simulink model "SoftGripperPick"  (R2026b)
settings: Solver=daessc  StopTime=16  RelTol=1e-4
undefined symbols (not defined in the file): magnitude, P, X, Y, Z
libraries: sm_lib x123, nesl_utility x40, fl_lib x4
(part 1 of 3)
settings Model: Creator=amavromm  LastModifiedBy=amavromm
settings SolverCC: ZeroCrossControl=DisableAll
settings SimscapeCC: SimscapeNominalValues="[{\"value\":\"1\",\"unit\":\"A\"},{\"value\":\"1\",\"unit\":\"bar\"},{\"value\":\"1\",\"unit\":\"cm^2\"},{\"value\":\"1\",\"unit\":\"cm^3/s\"},{\"value\":\"1\",\"unit\":\"kJ/kg\"},{\"value\":\"1\",\"unit\":\"kW\"},{\"value\":\"1\",\"unit\":\"l\"},{\"value\":\"1\",\"unit\":\"N\"},{\"value\":\"1\",\"unit\":\"N*m\"},{\"value\":\"1\",\"unit\":\"V\"},{\"value\":\"0.001\",\"unit\":\"Wb\"}]"  SimscapeUseEnergyAccounting=off

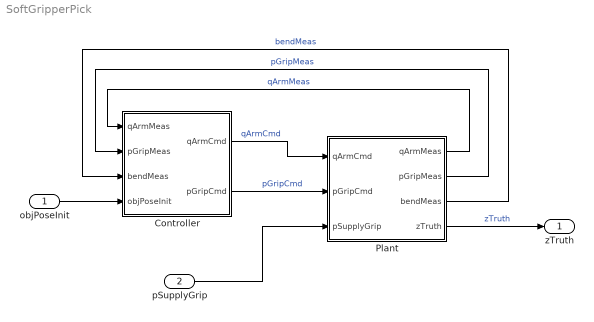
== system SoftGripperPick ==
  objPoseInit : Inport  PortDimensions=6
  pSupplyGrip : Inport  Port=2  PortDimensions=1
  Controller : Subsystem
  Plant : Subsystem
  zTruth : Outport
  wires:
  Plant/4(zTruth) -> zTruth/1  "zTruth"
  objPoseInit/1 -> Controller/4(objPoseInit)
  Plant/3(bendMeas) -> Controller/3(bendMeas)  "bendMeas"
  Plant/2(pGripMeas) -> Controller/2(pGripMeas)  "pGripMeas"
  Plant/1(qArmMeas) -> Controller/1(qArmMeas)  "qArmMeas"
  pSupplyGrip/1 -> Plant/3(pSupplyGrip)
  Controller/2(pGripCmd) -> Plant/2(pGripCmd)  "pGripCmd"
  Controller/1(qArmCmd) -> Plant/1(qArmCmd)  "qArmCmd"

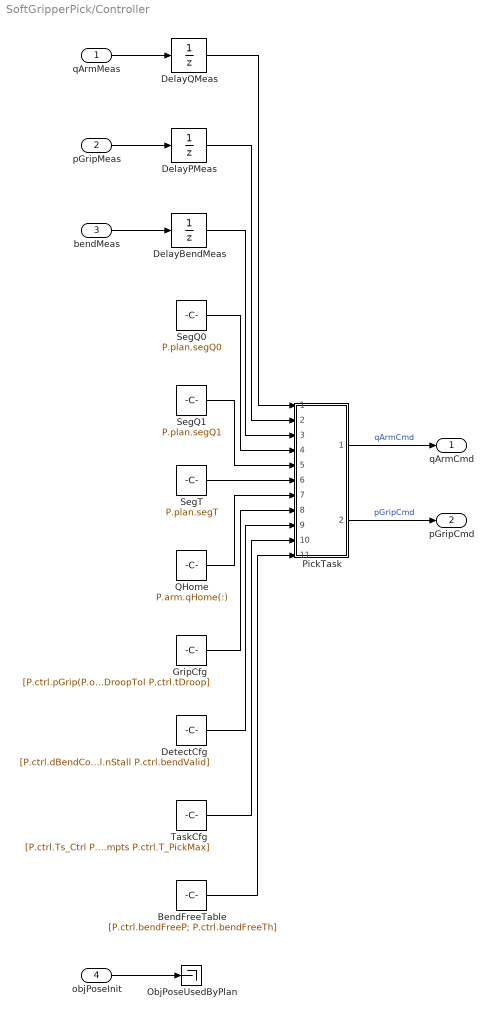
== system SoftGripperPick/Controller ==
  qArmMeas : Inport
  pGripMeas : Inport  Port=2
  bendMeas : Inport  Port=3
  objPoseInit : Inport  Port=4
  BendFreeTable : Constant  Value=[P.ctrl.bendFreeP; P.ctrl.bendFreeTh]
  DelayBendMeas : UnitDelay  InitialCondition=zeros(4,1)  SampleTime=P.ctrl.Ts_Ctrl
  DelayPMeas : UnitDelay  SampleTime=P.ctrl.Ts_Ctrl
  DelayQMeas : UnitDelay  InitialCondition=P.arm.qHome(:)  SampleTime=P.ctrl.Ts_Ctrl
  DetectCfg : Constant  Value=[P.ctrl.dBendContact P.ctrl.stallRate P.ctrl.nStall P.ctrl.bendValid]
  GripCfg : Constant  Value=[P.ctrl.pGrip(P.objId) P.ctrl.sens.pAcc P.ctrl.tCloseRamp P.ctrl.tCloseMax P.ctrl.tVent P.ctrl.pDroopTol P.ctrl.tDroop]
  ObjPoseUsedByPlan : Terminator
  PickTask : Stateflow chart  TreatAsAtomicUnit=on
  QHome : Constant  Value=P.arm.qHome(:)
  SegQ0 : Constant  Value=P.plan.segQ0
  SegQ1 : Constant  Value=P.plan.segQ1
  SegT : Constant  Value=P.plan.segT
  TaskCfg : Constant  Value=[P.ctrl.Ts_Ctrl P.ctrl.tSettle P.ctrl.qTol P.ctrl.N_Attempts P.ctrl.T_PickMax]
  qArmCmd : Outport
  pGripCmd : Outport  Port=2
  wires:
  DelayBendMeas/1 -> PickTask/3(bend)
  DelayPMeas/1 -> PickTask/2(pMeas)
  DelayQMeas/1 -> PickTask/1(qMeas)
  objPoseInit/1 -> ObjPoseUsedByPlan/1
  qArmMeas/1 -> DelayQMeas/1
  pGripMeas/1 -> DelayPMeas/1
  bendMeas/1 -> DelayBendMeas/1
  SegQ0/1 -> PickTask/4(segQ0)
  SegQ1/1 -> PickTask/5(segQ1)
  SegT/1 -> PickTask/6(segT)
  QHome/1 -> PickTask/7(qHome)
  GripCfg/1 -> PickTask/8(gripCfg)
  DetectCfg/1 -> PickTask/9(detCfg)
  TaskCfg/1 -> PickTask/10(taskCfg)
  BendFreeTable/1 -> PickTask/11(bendTab)
  PickTask/1(qCmd) -> qArmCmd/1  "qArmCmd"
  PickTask/2(pCmd) -> pGripCmd/1  "pGripCmd"

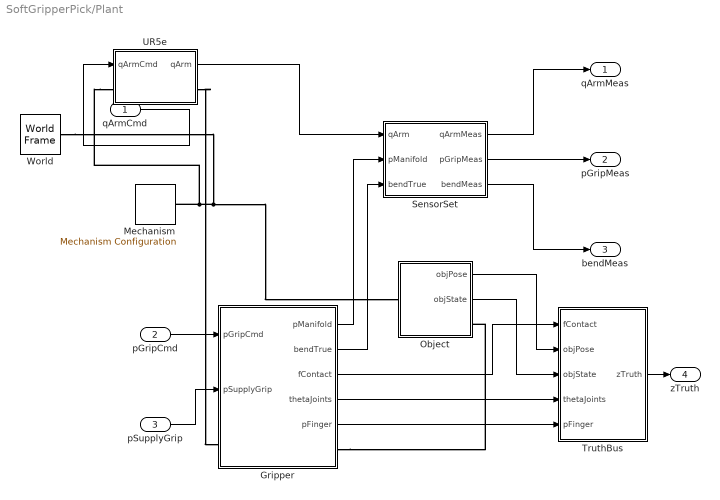
== system SoftGripperPick/Plant ==
  qArmCmd : Inport
  pGripCmd : Inport  Port=2
  pSupplyGrip : Inport  Port=3
  Gripper : Subsystem
  Mechanism : sm_lib/Utilities/Mechanism Configuration  UniformGravity=Constant  GravityVector=[0 0 -9.80665]  GravityVectorUnits=m/s^2  LinearizationDelta=0.001  JointModeTransitionNonlinearIterations=2
  Object : Subsystem
  SensorSet : Subsystem
  TruthBus : Subsystem
  UR5e : Subsystem
  World : sm_lib/Frames and Transforms/World Frame
  qArmMeas : Outport
  pGripMeas : Outport  Port=2
  bendMeas : Outport  Port=3
  zTruth : Outport  Port=4
  wires:
  Gripper/5(pFinger) -> TruthBus/5(pFinger)
  Gripper/4(thetaJoints) -> TruthBus/4(thetaJoints)
  Gripper/3(fContact) -> TruthBus/1(fContact)
  Gripper/2(bendTrue) -> SensorSet/3(bendTrue)
  Gripper/1(pManifold) -> SensorSet/2(pManifold)
  UR5e/1(qArm) -> SensorSet/1(qArm)
  pSupplyGrip/1 -> Gripper/2(pSupplyGrip)
  pGripCmd/1 -> Gripper/1(pGripCmd)
  qArmCmd/1 -> UR5e/1(qArmCmd)
  SensorSet/1(qArmMeas) -> qArmMeas/1
  SensorSet/2(pGripMeas) -> pGripMeas/1
  SensorSet/3(bendMeas) -> bendMeas/1
  Object/1(objPose) -> TruthBus/2(objPose)
  Object/2(objState) -> TruthBus/3(objState)
  TruthBus/1(zTruth) -> zTruth/1
  connections:
  UR5e/LConn1 -- World/RConn1 -- Object/LConn1 -- Mechanism/RConn1
  Gripper/RConn1 -- Object/RConn1
  UR5e/RConn1 -- Gripper/LConn1

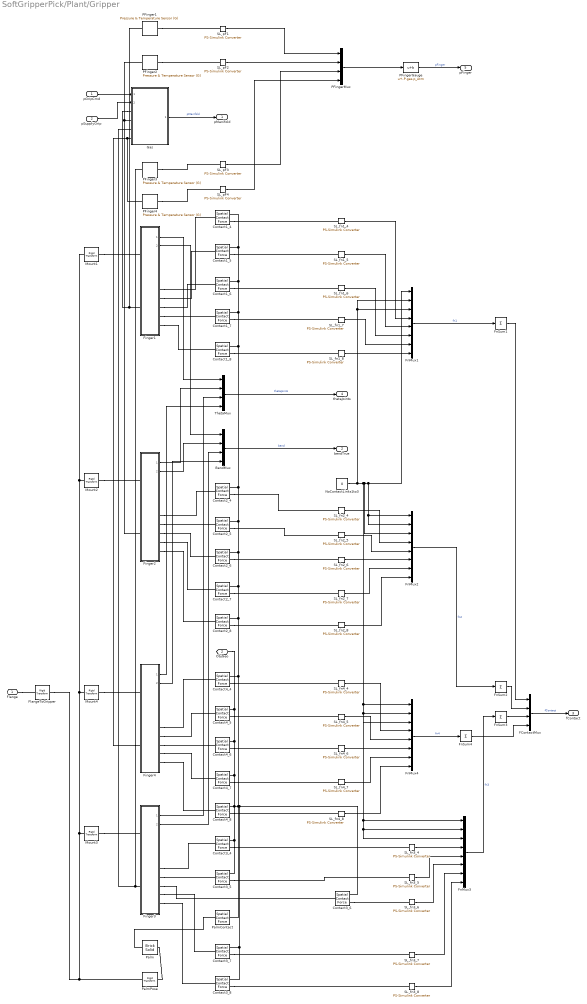
== system SoftGripperPick/Plant/Gripper ==
  pGripCmd : Inport
  pSupplyGrip : Inport  Port=2
  BendMux : Mux
  Contact1_{4..8} (5 alike) : sm_lib/Forces and Torques/Spatial Contact Force  SenseSeparationDistance=off  NormalForceType=SmoothSpringDamper  NormalStiffness=P.obj.k_Contact  NormalStiffnessUnits=N/m  NormalDamping=P.obj.c_Contact  NormalDampingUnits=N/(m/s)  NormalTransitionRegionWidth=P.bench.wContact  NormalTransitionRegionWidthUnits=m  FrictionType=SmoothStickSlip  CoefficientOfStaticFriction=P.obj.mu_s  CoefficientOfDynamicFriction=P.obj.mu_d  FrictionalCriticalVelocity=P.bench.vCrit  FrictionalCriticalVelocityUnits=m/s  SenseContactSignal=off  SensePenetrationDepth=off  SenseNormalVelocity=off  SenseTangentialVelocity=off  SensingForceTorqueDirection=BaseOnFollower  SensingForceTorqueResolutionFrame=ContactFrame  SenseNormalForce=off  SenseNormalForceMagnitude=on  SenseNormalTorque=off  SenseFrictionalForce=off  SenseFrictionalForceMagnitude=off  SenseFrictionalTorque=off  SenseTotalForce=off  SenseTotalTorque=off  SenseContactBaseRotation=off  SenseContactBaseTranslation=off  SenseContactFollowerRotation=off  SenseContactFollowerTranslation=off  ZeroCrossDetectContactStartAndEnd=off
  Contact2_{4..8} (5 alike) : sm_lib/Forces and Torques/Spatial Contact Force  SenseSeparationDistance=off  NormalForceType=SmoothSpringDamper  NormalStiffness=P.obj.k_Contact  NormalStiffnessUnits=N/m  NormalDamping=P.obj.c_Contact  NormalDampingUnits=N/(m/s)  NormalTransitionRegionWidth=P.bench.wContact  NormalTransitionRegionWidthUnits=m  FrictionType=SmoothStickSlip  CoefficientOfStaticFriction=P.obj.mu_s  CoefficientOfDynamicFriction=P.obj.mu_d  FrictionalCriticalVelocity=P.bench.vCrit  FrictionalCriticalVelocityUnits=m/s  SenseContactSignal=off  SensePenetrationDepth=off  SenseNormalVelocity=off  SenseTangentialVelocity=off  SensingForceTorqueDirection=BaseOnFollower  SensingForceTorqueResolutionFrame=ContactFrame  SenseNormalForce=off  SenseNormalForceMagnitude=on  SenseNormalTorque=off  SenseFrictionalForce=off  SenseFrictionalForceMagnitude=off  SenseFrictionalTorque=off  SenseTotalForce=off  SenseTotalTorque=off  SenseContactBaseRotation=off  SenseContactBaseTranslation=off  SenseContactFollowerRotation=off  SenseContactFollowerTranslation=off  ZeroCrossDetectContactStartAndEnd=off
  Contact3_{4..8} (5 alike) : sm_lib/Forces and Torques/Spatial Contact Force  SenseSeparationDistance=off  NormalForceType=SmoothSpringDamper  NormalStiffness=P.obj.k_Contact  NormalStiffnessUnits=N/m  NormalDamping=P.obj.c_Contact  NormalDampingUnits=N/(m/s)  NormalTransitionRegionWidth=P.bench.wContact  NormalTransitionRegionWidthUnits=m  FrictionType=SmoothStickSlip  CoefficientOfStaticFriction=P.obj.mu_s  CoefficientOfDynamicFriction=P.obj.mu_d  FrictionalCriticalVelocity=P.bench.vCrit  FrictionalCriticalVelocityUnits=m/s  SenseContactSignal=off  SensePenetrationDepth=off  SenseNormalVelocity=off  SenseTangentialVelocity=off  SensingForceTorqueDirection=BaseOnFollower  SensingForceTorqueResolutionFrame=ContactFrame  SenseNormalForce=off  SenseNormalForceMagnitude=on  SenseNormalTorque=off  SenseFrictionalForce=off  SenseFrictionalForceMagnitude=off  SenseFrictionalTorque=off  SenseTotalForce=off  SenseTotalTorque=off  SenseContactBaseRotation=off  SenseContactBaseTranslation=off  SenseContactFollowerRotation=off  SenseContactFollowerTranslation=off  ZeroCrossDetectContactStartAndEnd=off
  Contact4_{4..8} (5 alike) : sm_lib/Forces and Torques/Spatial Contact Force  SenseSeparationDistance=off  NormalForceType=SmoothSpringDamper  NormalStiffness=P.obj.k_Contact  NormalStiffnessUnits=N/m  NormalDamping=P.obj.c_Contact  NormalDampingUnits=N/(m/s)  NormalTransitionRegionWidth=P.bench.wContact  NormalTransitionRegionWidthUnits=m  FrictionType=SmoothStickSlip  CoefficientOfStaticFriction=P.obj.mu_s  CoefficientOfDynamicFriction=P.obj.mu_d  FrictionalCriticalVelocity=P.bench.vCrit  FrictionalCriticalVelocityUnits=m/s  SenseContactSignal=off  SensePenetrationDepth=off  SenseNormalVelocity=off  SenseTangentialVelocity=off  SensingForceTorqueDirection=BaseOnFollower  SensingForceTorqueResolutionFrame=ContactFrame  SenseNormalForce=off  SenseNormalForceMagnitude=on  SenseNormalTorque=off  SenseFrictionalForce=off  SenseFrictionalForceMagnitude=off  SenseFrictionalTorque=off  SenseTotalForce=off  SenseTotalTorque=off  SenseContactBaseRotation=off  SenseContactBaseTranslation=off  SenseContactFollowerRotation=off  SenseContactFollowerTranslation=off  ZeroCrossDetectContactStartAndEnd=off
  FContactMux : Mux
  Finger{1..4} (4 alike) : Subsystem  ReferencedSubsystem=SoftFinger
  FlangeToGripper : sm_lib/Frames and Transforms/Rigid Transform  RotationMethod=StandardAxis  FollAlignAxisA=+X  BaseAlignAxisA=+Y  FollAlignAxisB=+Y  BaseAlignAxisB=+Z  RotationStandardAxis=+X  RotationAngle=180  RotationAngleUnits=deg  RotationArbitraryAxis=[0 0 1]  RotationSequenceAxes=FollowerAxes  RotationSequence=XYX  RotationSequenceAngles=[0 0 0]  RotationSequenceAnglesUnits=deg  RotationMatrix=[1 0 0;0 1 0;0 0 1]  Quaternion=[1 0 0 0]  TranslationMethod=None  TranslationCartesianOffset=[0 0 0]  TranslationCartesianOffsetUnits=m  TranslationStandardAxis=+Z  TranslationStandardOffset=0  TranslationStandardOffsetUnits=m  TranslationROffset=0  TranslationROffsetUnits=m  TranslationThetaOffset=0  TranslationThetaOffsetUnits=deg  TranslationZOffset=0  TranslationZOffsetUnits=m
  FnMux{1..4} (4 alike) : Mux  Inputs=8
  FnSum{1..4} (4 alike) : Sum  Inputs=+
  Gas : Subsystem  ReferencedSubsystem=GripperGas
  Mount1 : sm_lib/Frames and Transforms/Rigid Transform  RotationMethod=RotationMatrix  FollAlignAxisA=+X  BaseAlignAxisA=+Y  FollAlignAxisB=+Y  BaseAlignAxisB=+Z  RotationStandardAxis=+Z  RotationAngle=0  RotationAngleUnits=deg  RotationArbitraryAxis=[0 0 1]  RotationSequenceAxes=FollowerAxes  RotationSequence=XYX  RotationSequenceAngles=[0 0 0]  RotationSequenceAnglesUnits=deg  RotationMatrix=P.bench.mountR(:,:,1)  Quaternion=[1 0 0 0]  TranslationMethod=Cartesian  TranslationCartesianOffset=P.bench.mountT(1,:)  TranslationCartesianOffsetUnits=m  TranslationStandardAxis=+Z  TranslationStandardOffset=0  TranslationStandardOffsetUnits=m  TranslationROffset=0  TranslationROffsetUnits=m  TranslationThetaOffset=0  TranslationThetaOffsetUnits=deg  TranslationZOffset=0  TranslationZOffsetUnits=m
  Mount2 : sm_lib/Frames and Transforms/Rigid Transform  RotationMethod=RotationMatrix  FollAlignAxisA=+X  BaseAlignAxisA=+Y  FollAlignAxisB=+Y  BaseAlignAxisB=+Z  RotationStandardAxis=+Z  RotationAngle=0  RotationAngleUnits=deg  RotationArbitraryAxis=[0 0 1]  RotationSequenceAxes=FollowerAxes  RotationSequence=XYX  RotationSequenceAngles=[0 0 0]  RotationSequenceAnglesUnits=deg  RotationMatrix=P.bench.mountR(:,:,2)  Quaternion=[1 0 0 0]  TranslationMethod=Cartesian  TranslationCartesianOffset=P.bench.mountT(2,:)  TranslationCartesianOffsetUnits=m  TranslationStandardAxis=+Z  TranslationStandardOffset=0  TranslationStandardOffsetUnits=m  TranslationROffset=0  TranslationROffsetUnits=m  TranslationThetaOffset=0  TranslationThetaOffsetUnits=deg  TranslationZOffset=0  TranslationZOffsetUnits=m
  Mount3 : sm_lib/Frames and Transforms/Rigid Transform  RotationMethod=RotationMatrix  FollAlignAxisA=+X  BaseAlignAxisA=+Y  FollAlignAxisB=+Y  BaseAlignAxisB=+Z  RotationStandardAxis=+Z  RotationAngle=0  RotationAngleUnits=deg  RotationArbitraryAxis=[0 0 1]  RotationSequenceAxes=FollowerAxes  RotationSequence=XYX  RotationSequenceAngles=[0 0 0]  RotationSequenceAnglesUnits=deg  RotationMatrix=P.bench.mountR(:,:,3)  Quaternion=[1 0 0 0]  TranslationMethod=Cartesian  TranslationCartesianOffset=P.bench.mountT(3,:)  TranslationCartesianOffsetUnits=m  TranslationStandardAxis=+Z  TranslationStandardOffset=0  TranslationStandardOffsetUnits=m  TranslationROffset=0  TranslationROffsetUnits=m  TranslationThetaOffset=0  TranslationThetaOffsetUnits=deg  TranslationZOffset=0  TranslationZOffsetUnits=m
  Mount4 : sm_lib/Frames and Transforms/Rigid Transform  RotationMethod=RotationMatrix  FollAlignAxisA=+X  BaseAlignAxisA=+Y  FollAlignAxisB=+Y  BaseAlignAxisB=+Z  RotationStandardAxis=+Z  RotationAngle=0  RotationAngleUnits=deg  RotationArbitraryAxis=[0 0 1]  RotationSequenceAxes=FollowerAxes  RotationSequence=XYX  RotationSequenceAngles=[0 0 0]  RotationSequenceAnglesUnits=deg  RotationMatrix=P.bench.mountR(:,:,4)  Quaternion=[1 0 0 0]  TranslationMethod=Cartesian  TranslationCartesianOffset=P.bench.mountT(4,:)  TranslationCartesianOffsetUnits=m  TranslationStandardAxis=+Z  TranslationStandardOffset=0  TranslationStandardOffsetUnits=m  TranslationROffset=0  TranslationROffsetUnits=m  TranslationThetaOffset=0  TranslationThetaOffsetUnits=deg  TranslationZOffset=0  TranslationZOffsetUnits=m
  NoContactLinks1to3 : Constant  Value=0
  PFinger{1..4} (4 alike) : fl_lib/Gas/Sensors/Pressure & Temperature Sensor (G)  reference=foundation.enum.MeasurementReference.absolute  pressure=true  pressure_spec=foundation.enum.PressureMeasementSpec.Absolute  temperature=false
  PFingerGauge : Bias  Bias=-P.gas.p_Atm  SaturateOnIntegerOverflow=off
  PFingerMux : Mux
  Palm : sm_lib/Body Elements/Brick Solid  BrickDimensions=[P.bench.wPalm P.bench.wPalm P.bench.tPalm]  BrickDimensionsUnits=m  ExportEntireGeometry=on  InertiaType=CalculateFromGeometry  BasedOnType=Density  Density=1000  DensityUnits=kg/m^3  Mass=1  MassUnits=kg  CenterOfMass=[0 0 0]  CenterOfMassUnits=m  MomentsOfInertia=[1 1 1]  MomentsOfInertiaUnits=kg*m^2  ProductsOfInertia=[0 0 0]  ProductsOfInertiaUnits=kg*m^2  GraphicType=FromGeometry  MarkerShape=Sphere  MarkerSize=10  GraphicVisPropType=SimpleVisualProperties  GraphicDiffuseColor=[0.7 0.7 0.75]  GraphicOpacity=1  GraphicSpecularColor=[0.5 0.5 0.5 1.0]  GraphicAmbientColor=[0.15 0.15 0.15 1.0]  GraphicEmissiveColor=[0.0 0.0 0.0 1.0]  GraphicShininess=75  DoExposeReferenceFrame=on  SerializedFrames=<Frames/>
  PalmContact : sm_lib/Forces and Torques/Spatial Contact Force  SenseSeparationDistance=off  NormalForceType=SmoothSpringDamper  NormalStiffness=P.obj.k_Table  NormalStiffnessUnits=N/m  NormalDamping=P.obj.c_Table  NormalDampingUnits=N/(m/s)  NormalTransitionRegionWidth=P.bench.wContact  NormalTransitionRegionWidthUnits=m  FrictionType=SmoothStickSlip  CoefficientOfStaticFriction=P.obj.mu_s  CoefficientOfDynamicFriction=P.obj.mu_d  FrictionalCriticalVelocity=P.bench.vCrit  FrictionalCriticalVelocityUnits=m/s  SenseContactSignal=off  SensePenetrationDepth=off  SenseNormalVelocity=off  SenseTangentialVelocity=off  SensingForceTorqueDirection=BaseOnFollower  SensingForceTorqueResolutionFrame=ContactFrame  SenseNormalForce=off  SenseNormalForceMagnitude=off  SenseNormalTorque=off  SenseFrictionalForce=off  SenseFrictionalForceMagnitude=off  SenseFrictionalTorque=off  SenseTotalForce=off  SenseTotalTorque=off  SenseContactBaseRotation=off  SenseContactBaseTranslation=off  SenseContactFollowerRotation=off  SenseContactFollowerTranslation=off  ZeroCrossDetectContactStartAndEnd=off
  PalmPose : sm_lib/Frames and Transforms/Rigid Transform  RotationMethod=None  FollAlignAxisA=+X  BaseAlignAxisA=+Y  FollAlignAxisB=+Y  BaseAlignAxisB=+Z  RotationStandardAxis=+Z  RotationAngle=0  RotationAngleUnits=deg  RotationArbitraryAxis=[0 0 1]  RotationSequenceAxes=FollowerAxes  RotationSequence=XYX  RotationSequenceAngles=[0 0 0]  RotationSequenceAnglesUnits=deg  RotationMatrix=[1 0 0;0 1 0;0 0 1]  Quaternion=[1 0 0 0]  TranslationMethod=Cartesian  TranslationCartesianOffset=[0 0 P.bench.tPalm/2]  TranslationCartesianOffsetUnits=m  TranslationStandardAxis=+Z  TranslationStandardOffset=0  TranslationStandardOffsetUnits=m  TranslationROffset=0  TranslationROffsetUnits=m  TranslationThetaOffset=0  TranslationThetaOffsetUnits=deg  TranslationZOffset=0  TranslationZOffsetUnits=m
  SL_fn1_{4..8} (5 alike) : nesl_utility/PS-Simulink Converter  PhysicalDomain=network_engine_domain  SubClassName=ps_output  LeftPortType=input  RightPortType=output  PseudoPeriodic=off  Frequencies=[]  VectorFormat=inherit  Unit=N  AffineConversion=off
  SL_fn2_{4..8} (5 alike) : nesl_utility/PS-Simulink Converter  PhysicalDomain=network_engine_domain  SubClassName=ps_output  LeftPortType=input  RightPortType=output  PseudoPeriodic=off  Frequencies=[]  VectorFormat=inherit  Unit=N  AffineConversion=off
  SL_fn3_{4..8} (5 alike) : nesl_utility/PS-Simulink Converter  PhysicalDomain=network_engine_domain  SubClassName=ps_output  LeftPortType=input  RightPortType=output  PseudoPeriodic=off  Frequencies=[]  VectorFormat=inherit  Unit=N  AffineConversion=off
  SL_fn4_{4..8} (5 alike) : nesl_utility/PS-Simulink Converter  PhysicalDomain=network_engine_domain  SubClassName=ps_output  LeftPortType=input  RightPortType=output  PseudoPeriodic=off  Frequencies=[]  VectorFormat=inherit  Unit=N  AffineConversion=off
  SL_pF{1..4} (4 alike) : nesl_utility/PS-Simulink Converter  PhysicalDomain=network_engine_domain  SubClassName=ps_output  LeftPortType=input  RightPortType=output  PseudoPeriodic=off  Frequencies=[]  VectorFormat=inherit  Unit=Pa  AffineConversion=off
  ThetaMux : Mux
  Flange : PMIOPort  Side=Left
  ObjGeo : PMIOPort  Port=2  Side=Right
  pManifold : Outport
  bendTrue : Outport  Port=2
  fContact : Outport  Port=3
  thetaJoints : Outport  Port=4
  pFinger : Outport  Port=5
  wires:
  NoContactLinks1to3/1 -> FnMux4/2, FnMux4/3, FnMux4/1, FnMux3/3, FnMux3/2, FnMux3/1, FnMux2/1, FnMux2/2, FnMux1/1, FnMux2/3, FnMux1/3, FnMux1/2
  SL_fn4_8/1 -> FnMux4/8
  SL_fn4_7/1 -> FnMux4/7
  SL_fn4_6/1 -> FnMux4/6
  SL_fn4_5/1 -> FnMux4/5
  SL_fn4_4/1 -> FnMux4/4
  SL_fn2_8/1 -> FnMux2/8
  SL_fn2_7/1 -> FnMux2/7
  SL_fn2_6/1 -> FnMux2/6
  SL_fn2_5/1 -> FnMux2/5
  SL_fn2_4/1 -> FnMux2/4
  SL_fn1_8/1 -> FnMux1/8
  SL_fn1_7/1 -> FnMux1/7
  SL_fn1_6/1 -> FnMux1/6
  SL_fn1_5/1 -> FnMux1/5
  SL_fn1_4/1 -> FnMux1/4
  pGripCmd/1 -> Gas/1
  Gas/1 -> pManifold/1  "pManifold"
  Finger1/2 -> BendMux/1
  Finger2/2 -> BendMux/2
  Finger3/2 -> BendMux/3
  Finger4/2 -> BendMux/4
  BendMux/1 -> bendTrue/1  "bend"
  SL_fn3_4/1 -> FnMux3/4
  SL_fn3_5/1 -> FnMux3/5
  SL_fn3_6/1 -> FnMux3/6
  SL_fn3_7/1 -> FnMux3/7
  SL_fn3_8/1 -> FnMux3/8
  pSupplyGrip/1 -> Gas/2
  FnMux1/1 -> FnSum1/1  "fn1"
  FnMux2/1 -> FnSum2/1  "fn2"
  FnMux3/1 -> FnSum3/1  "fn3"
  FnMux4/1 -> FnSum4/1  "fn4"
  FnSum1/1 -> FContactMux/1
  FnSum2/1 -> FContactMux/2
  FnSum3/1 -> FContactMux/3
  FnSum4/1 -> FContactMux/4
  FContactMux/1 -> fContact/1  "fContact"
  Finger1/1 -> ThetaMux/1
  Finger2/1 -> ThetaMux/2
  Finger3/1 -> ThetaMux/3
  Finger4/1 -> ThetaMux/4
  ThetaMux/1 -> thetaJoints/1  "thetaJoints"
  SL_pF1/1 -> PFingerMux/1
  SL_pF2/1 -> PFingerMux/2
  SL_pF3/1 -> PFingerMux/3
  SL_pF4/1 -> PFingerMux/4
  PFingerMux/1 -> PFingerGauge/1
  PFingerGauge/1 -> pFinger/1  "pFinger"
  connections:
  Contact3_6/RConn1 -- Contact3_8/RConn1 -- Contact3_7/RConn1 -- Contact1_4/RConn1 -- Contact1_5/RConn1 -- Contact1_6/RConn1 -- Contact1_7/RConn1 -- Contact1_8/RConn1 -- Contact2_4/RConn1 -- Contact2_5/RConn1 -- Contact2_6/RConn1 -- Contact2_7/RConn1 -- Contact2_8/RConn1 -- Contact4_4/RConn1 -- Contact3_4/RConn1 -- Contact3_5/RConn1 -- ObjGeo/RConn1 -- Contact4_5/RConn1 -- Contact4_6/RConn1 -- Contact4_7/RConn1 -- Contact4_8/RConn1 -- PalmContact/RConn1
  FlangeToGripper/RConn1 -- Mount1/LConn1 -- Mount2/LConn1 -- Mount4/LConn1 -- Mount3/LConn1 -- PalmPose/LConn1
  Palm/LConn1 -- PalmContact/LConn1
  PalmPose/RConn1 -- Palm/RConn1
  Mount4/RConn1 -- Finger4/LConn1
  Mount3/RConn1 -- Finger3/LConn1
  Mount2/RConn1 -- Finger2/LConn1
  Mount1/RConn1 -- Finger1/LConn1
  Finger4/RConn9 -- Contact4_8/LConn1
  Finger4/RConn8 -- Contact4_7/LConn1
  Finger4/RConn7 -- Contact4_6/LConn1
  Finger4/RConn6 -- Contact4_5/LConn1
  Finger4/RConn5 -- Contact4_4/LConn1
  Finger3/RConn9 -- Contact3_8/LConn1
  Finger3/RConn8 -- Contact3_7/LConn1
  Finger3/RConn7 -- Contact3_6/LConn1
  Finger3/RConn6 -- Contact3_5/LConn1
  Finger3/RConn5 -- Contact3_4/LConn1
  Finger2/RConn9 -- Contact2_8/LConn1
  Finger2/RConn8 -- Contact2_7/LConn1
  Finger2/RConn7 -- Contact2_6/LConn1
  Finger2/RConn6 -- Contact2_5/LConn1
  Finger2/RConn5 -- Contact2_4/LConn1
  Finger1/RConn9 -- Contact1_8/LConn1
  Finger1/RConn8 -- Contact1_7/LConn1
  Finger1/RConn7 -- Contact1_6/LConn1
  Finger1/RConn6 -- Contact1_5/LConn1
  Finger1/RConn5 -- Contact1_4/LConn1
  Gas/LConn1 -- Finger1/LConn2 -- PFinger1/LConn1
  PFinger2/LConn1 -- Finger2/LConn2 -- Gas/LConn2
  Finger3/LConn2 -- PFinger3/LConn1 -- Gas/LConn3
  Finger4/LConn2 -- PFinger4/LConn1 -- Gas/LConn4
  Flange/RConn1 -- FlangeToGripper/LConn1
  PFinger1/RConn1 -- SL_pF1/LConn1
  PFinger2/RConn1 -- SL_pF2/LConn1
  PFinger3/RConn1 -- SL_pF3/LConn1
  PFinger4/RConn1 -- SL_pF4/LConn1
  Contact1_4/RConn2 -- SL_fn1_4/LConn1
  Contact1_5/RConn2 -- SL_fn1_5/LConn1
  Contact1_6/RConn2 -- SL_fn1_6/LConn1
  Contact1_7/RConn2 -- SL_fn1_7/LConn1
  Contact1_8/RConn2 -- SL_fn1_8/LConn1
  Contact2_4/RConn2 -- SL_fn2_4/LConn1
  Contact2_5/RConn2 -- SL_fn2_5/LConn1
  Contact2_6/RConn2 -- SL_fn2_6/LConn1
  Contact2_7/RConn2 -- SL_fn2_7/LConn1
  Contact2_8/RConn2 -- SL_fn2_8/LConn1
  Contact3_4/RConn2 -- SL_fn3_4/LConn1
  Contact3_5/RConn2 -- SL_fn3_5/LConn1
  Contact3_6/RConn2 -- SL_fn3_6/LConn1
  Contact3_7/RConn2 -- SL_fn3_7/LConn1
  Contact3_8/RConn2 -- SL_fn3_8/LConn1
  Contact4_4/RConn2 -- SL_fn4_4/LConn1
  Contact4_5/RConn2 -- SL_fn4_5/LConn1
  Contact4_6/RConn2 -- SL_fn4_6/LConn1
  Contact4_7/RConn2 -- SL_fn4_7/LConn1
  Contact4_8/RConn2 -- SL_fn4_8/LConn1

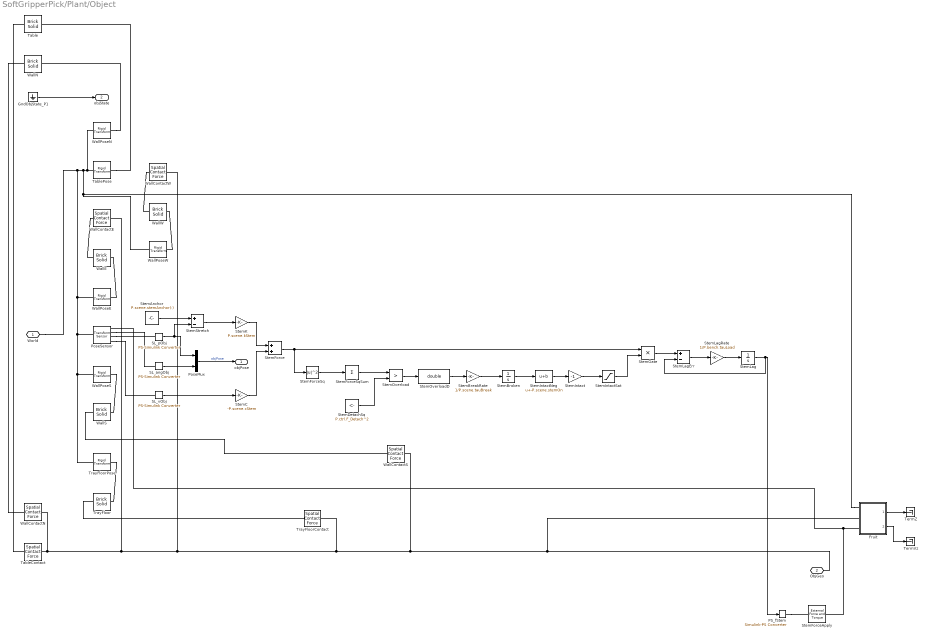
== system SoftGripperPick/Plant/Object ==
  Fruit : Subsystem  ReferencedSubsystem=ObjectBody
  GndObjState_P1 : Ground
  PS_fStem : nesl_utility/Simulink-PS Converter  PhysicalDomain=network_engine_domain  SubClassName=ps_input  LeftPortType=input  RightPortType=output  PseudoPeriodic=off  Frequencies=[]  NoiseDistribution=none  NoiseParameters=[]  Unit=N  AffineConversion=off  FilteringAndDerivatives=provide  SimscapeFilterOrder=1  InputFilterTimeConstant=0.001  UdotUserProvided=0
  PoseMux : Mux  Inputs=2
  PoseSensor : sm_lib/Frames and Transforms/Transform Sensor  ObservationFrame=World  ExpressedInFrame=World  RotationSequence=XYX  SenseAngle=off  SenseAxis=off  SenseQ=off  SenseR=off  SenseRotationSequence=on  SenseOmegaX=off  SenseOmegaY=off  SenseOmegaZ=off  SenseOmega=off  SenseQDot=off  SenseRDot=off  SenseRotationSequenceDot=off  SenseAlphaX=off  SenseAlphaY=off  SenseAlphaZ=off  SenseAlpha=off  SenseQDDot=off  SenseRDDot=off  SenseX=off  SenseY=off  SenseZ=off  SenseXYZ=on  SenseRad=off  SenseAzim=off  SenseDist=off  SenseInc=off  SenseXDot=off  SenseYDot=off  SenseZDot=off  SenseXYZDot=on  SenseRadDot=off  SenseAzimDot=off  SenseDistDot=off  SenseIncDot=off  SenseXDDot=off  SenseYDDot=off  SenseZDDot=off  SenseXYZDDot=off  SenseRadDDot=off  SenseAzimDDot=off  SenseDistDDot=off  SenseIncDDot=off
  SL_angObj : nesl_utility/PS-Simulink Converter  PhysicalDomain=network_engine_domain  SubClassName=ps_output  LeftPortType=input  RightPortType=output  PseudoPeriodic=off  Frequencies=[]  VectorFormat=inherit  Unit=rad  AffineConversion=off
  SL_pObj : nesl_utility/PS-Simulink Converter  PhysicalDomain=network_engine_domain  SubClassName=ps_output  LeftPortType=input  RightPortType=output  PseudoPeriodic=off  Frequencies=[]  VectorFormat=inherit  Unit=m  AffineConversion=off
  SL_vObj : nesl_utility/PS-Simulink Converter  PhysicalDomain=network_engine_domain  SubClassName=ps_output  LeftPortType=input  RightPortType=output  PseudoPeriodic=off  Frequencies=[]  VectorFormat=inherit  Unit=m/s  AffineConversion=off
  StemAnchor : Constant  Value=P.scene.stemAnchor(:)
  StemBreakRate : Gain  Gain=1/P.scene.tauBreak
  StemBroken : Integrator  LimitOutput=on  UpperSaturationLimit=1  LowerSaturationLimit=0
  StemC : Gain  Gain=-P.scene.cStem
  StemDetachSq : Constant  Value=P.ctrl.F_Detach^2
  StemForce : Sum
  StemForceApply : sm_lib/Forces and Torques/External Force and Torque  EnableForceX=off  EnableForceY=off  EnableForceZ=off  EnableForce=on  ForceResolutionFrame=World  EnableTorqueX=off  EnableTorqueY=off  EnableTorqueZ=off  EnableTorque=off  TorqueResolutionFrame=AttachedFrame
  StemForceSq : Math  Operator=magnitude^2
  StemForceSqSum : Sum  Inputs=+
  StemGate : Product
  StemIntact : Gain  Gain=-1
  StemIntactNeg : Bias  Bias=-P.scene.stemOn  SaturateOnIntegerOverflow=off
  StemIntactSat : Saturate  UpperLimit=1  LowerLimit=0
  StemK : Gain  Gain=P.scene.kStem
  StemLag : Integrator  InitialCondition=zeros(3,1)
  StemLagErr : Sum  Inputs=+-
  StemLagRate : Gain  Gain=1/P.bench.tauLoad
  StemOverload : RelationalOperator  Operator=>  OutDataTypeStr=boolean  RndMeth=Simplest  InputSameDT=off
  StemOverloadD : DataTypeConversion  OutDataTypeStr=double  SaturateOnIntegerOverflow=off  RndMeth=Floor
  StemStretch : Sum  Inputs=+-
  Table : sm_lib/Body Elements/Brick Solid  BrickDimensions=[P.scene.wTable P.scene.wTable P.scene.tTable]  BrickDimensionsUnits=m  ExportEntireGeometry=on  InertiaType=CalculateFromGeometry  BasedOnType=Density  Density=1000  DensityUnits=kg/m^3  Mass=1  MassUnits=kg  CenterOfMass=[0 0 0]  CenterOfMassUnits=m  MomentsOfInertia=[1 1 1]  MomentsOfInertiaUnits=kg*m^2  ProductsOfInertia=[0 0 0]  ProductsOfInertiaUnits=kg*m^2  GraphicType=FromGeometry  MarkerShape=Sphere  MarkerSize=10  GraphicVisPropType=SimpleVisualProperties  GraphicDiffuseColor=[0.6 0.45 0.3]  GraphicOpacity=1  GraphicSpecularColor=[0.5 0.5 0.5 1.0]  GraphicAmbientColor=[0.15 0.15 0.15 1.0]  GraphicEmissiveColor=[0.0 0.0 0.0 1.0]  GraphicShininess=75  DoExposeReferenceFrame=on  SerializedFrames=<Frames/>
  TableContact : sm_lib/Forces and Torques/Spatial Contact Force  SenseSeparationDistance=off  NormalForceType=SmoothSpringDamper  NormalStiffness=P.obj.k_Table  NormalStiffnessUnits=N/m  NormalDamping=P.obj.c_Table  NormalDampingUnits=N/(m/s)  NormalTransitionRegionWidth=P.bench.wContact  NormalTransitionRegionWidthUnits=m  FrictionType=SmoothStickSlip  CoefficientOfStaticFriction=P.obj.mu_s  CoefficientOfDynamicFriction=P.obj.mu_d  FrictionalCriticalVelocity=P.bench.vCrit  FrictionalCriticalVelocityUnits=m/s  SenseContactSignal=off  SensePenetrationDepth=off  SenseNormalVelocity=off  SenseTangentialVelocity=off  SensingForceTorqueDirection=BaseOnFollower  SensingForceTorqueResolutionFrame=ContactFrame  SenseNormalForce=off  SenseNormalForceMagnitude=off  SenseNormalTorque=off  SenseFrictionalForce=off  SenseFrictionalForceMagnitude=off  SenseFrictionalTorque=off  SenseTotalForce=off  SenseTotalTorque=off  SenseContactBaseRotation=off  SenseContactBaseTranslation=off  SenseContactFollowerRotation=off  SenseContactFollowerTranslation=off  ZeroCrossDetectContactStartAndEnd=off
  TablePose : sm_lib/Frames and Transforms/Rigid Transform  RotationMethod=None  FollAlignAxisA=+X  BaseAlignAxisA=+Y  FollAlignAxisB=+Y  BaseAlignAxisB=+Z  RotationStandardAxis=+Z  RotationAngle=0  RotationAngleUnits=deg  RotationArbitraryAxis=[0 0 1]  RotationSequenceAxes=FollowerAxes  RotationSequence=XYX  RotationSequenceAngles=[0 0 0]  RotationSequenceAnglesUnits=deg  RotationMatrix=[1 0 0;0 1 0;0 0 1]  Quaternion=[1 0 0 0]  TranslationMethod=Cartesian  TranslationCartesianOffset=[P.scene.tableXY -P.scene.tTable/2]  TranslationCartesianOffsetUnits=m  TranslationStandardAxis=+Z  TranslationStandardOffset=0  TranslationStandardOffsetUnits=m  TranslationROffset=0  TranslationROffsetUnits=m  TranslationThetaOffset=0  TranslationThetaOffsetUnits=deg  TranslationZOffset=0  TranslationZOffsetUnits=m
  TermVz : Terminator
  TermZ : Terminator
  TrayFloor : sm_lib/Body Elements/Brick Solid  BrickDimensions=[P.scene.wTray P.scene.wTray P.scene.trayZ]  BrickDimensionsUnits=m  ExportEntireGeometry=on  InertiaType=CalculateFromGeometry  BasedOnType=Density  Density=1000  DensityUnits=kg/m^3  Mass=1  MassUnits=kg  CenterOfMass=[0 0 0]  CenterOfMassUnits=m  MomentsOfInertia=[1 1 1]  MomentsOfInertiaUnits=kg*m^2  ProductsOfInertia=[0 0 0]  ProductsOfInertiaUnits=kg*m^2  GraphicType=FromGeometry  MarkerShape=Sphere  MarkerSize=10  GraphicVisPropType=SimpleVisualProperties  GraphicDiffuseColor=[0.2 0.35 0.6]  GraphicOpacity=1  GraphicSpecularColor=[0.5 0.5 0.5 1.0]  GraphicAmbientColor=[0.15 0.15 0.15 1.0]  GraphicEmissiveColor=[0.0 0.0 0.0 1.0]  GraphicShininess=75  DoExposeReferenceFrame=on  SerializedFrames=<Frames/>
  TrayFloorContact : sm_lib/Forces and Torques/Spatial Contact Force  SenseSeparationDistance=off  NormalForceType=SmoothSpringDamper  NormalStiffness=P.obj.k_Table  NormalStiffnessUnits=N/m  NormalDamping=P.obj.c_Table  NormalDampingUnits=N/(m/s)  NormalTransitionRegionWidth=P.bench.wContact  NormalTransitionRegionWidthUnits=m  FrictionType=SmoothStickSlip  CoefficientOfStaticFriction=P.obj.mu_s  CoefficientOfDynamicFriction=P.obj.mu_d  FrictionalCriticalVelocity=P.bench.vCrit  FrictionalCriticalVelocityUnits=m/s  SenseContactSignal=off  SensePenetrationDepth=off  SenseNormalVelocity=off  SenseTangentialVelocity=off  SensingForceTorqueDirection=BaseOnFollower  SensingForceTorqueResolutionFrame=ContactFrame  SenseNormalForce=off  SenseNormalForceMagnitude=off  SenseNormalTorque=off  SenseFrictionalForce=off  SenseFrictionalForceMagnitude=off  SenseFrictionalTorque=off  SenseTotalForce=off  SenseTotalTorque=off  SenseContactBaseRotation=off  SenseContactBaseTranslation=off  SenseContactFollowerRotation=off  SenseContactFollowerTranslation=off  ZeroCrossDetectContactStartAndEnd=off
  TrayFloorPose : sm_lib/Frames and Transforms/Rigid Transform  RotationMethod=None  FollAlignAxisA=+X  BaseAlignAxisA=+Y  FollAlignAxisB=+Y  BaseAlignAxisB=+Z  RotationStandardAxis=+Z  RotationAngle=0  RotationAngleUnits=deg  RotationArbitraryAxis=[0 0 1]  RotationSequenceAxes=FollowerAxes  RotationSequence=XYX  RotationSequenceAngles=[0 0 0]  RotationSequenceAnglesUnits=deg  RotationMatrix=[1 0 0;0 1 0;0 0 1]  Quaternion=[1 0 0 0]  TranslationMethod=Cartesian  TranslationCartesianOffset=[P.scene.trayXY P.scene.trayZ/2]  TranslationCartesianOffsetUnits=m  TranslationStandardAxis=+Z  TranslationStandardOffset=0  TranslationStandardOffsetUnits=m  TranslationROffset=0  TranslationROffsetUnits=m  TranslationThetaOffset=0  TranslationThetaOffsetUnits=deg  TranslationZOffset=0  TranslationZOffsetUnits=m
  WallContactE : sm_lib/Forces and Torques/Spatial Contact Force  SenseSeparationDistance=off  NormalForceType=SmoothSpringDamper  NormalStiffness=P.obj.k_Table  NormalStiffnessUnits=N/m  NormalDamping=P.obj.c_Table  NormalDampingUnits=N/(m/s)  NormalTransitionRegionWidth=P.bench.wContact  NormalTransitionRegionWidthUnits=m  FrictionType=SmoothStickSlip  CoefficientOfStaticFriction=P.obj.mu_s  CoefficientOfDynamicFriction=P.obj.mu_d  FrictionalCriticalVelocity=P.bench.vCrit  FrictionalCriticalVelocityUnits=m/s  SenseContactSignal=off  SensePenetrationDepth=off  SenseNormalVelocity=off  SenseTangentialVelocity=off  SensingForceTorqueDirection=BaseOnFollower  SensingForceTorqueResolutionFrame=ContactFrame  SenseNormalForce=off  SenseNormalForceMagnitude=off  SenseNormalTorque=off  SenseFrictionalForce=off  SenseFrictionalForceMagnitude=off  SenseFrictionalTorque=off  SenseTotalForce=off  SenseTotalTorque=off  SenseContactBaseRotation=off  SenseContactBaseTranslation=off  SenseContactFollowerRotation=off  SenseContactFollowerTranslation=off  ZeroCrossDetectContactStartAndEnd=off
  WallContactN : sm_lib/Forces and Torques/Spatial Contact Force  SenseSeparationDistance=off  NormalForceType=SmoothSpringDamper  NormalStiffness=P.obj.k_Table  NormalStiffnessUnits=N/m  NormalDamping=P.obj.c_Table  NormalDampingUnits=N/(m/s)  NormalTransitionRegionWidth=P.bench.wContact  NormalTransitionRegionWidthUnits=m  FrictionType=SmoothStickSlip  CoefficientOfStaticFriction=P.obj.mu_s  CoefficientOfDynamicFriction=P.obj.mu_d  FrictionalCriticalVelocity=P.bench.vCrit  FrictionalCriticalVelocityUnits=m/s  SenseContactSignal=off  SensePenetrationDepth=off  SenseNormalVelocity=off  SenseTangentialVelocity=off  SensingForceTorqueDirection=BaseOnFollower  SensingForceTorqueResolutionFrame=ContactFrame  SenseNormalForce=off  SenseNormalForceMagnitude=off  SenseNormalTorque=off  SenseFrictionalForce=off  SenseFrictionalForceMagnitude=off  SenseFrictionalTorque=off  SenseTotalForce=off  SenseTotalTorque=off  SenseContactBaseRotation=off  SenseContactBaseTranslation=off  SenseContactFollowerRotation=off  SenseContactFollowerTranslation=off  ZeroCrossDetectContactStartAndEnd=off
  WallContactS : sm_lib/Forces and Torques/Spatial Contact Force  SenseSeparationDistance=off  NormalForceType=SmoothSpringDamper  NormalStiffness=P.obj.k_Table  NormalStiffnessUnits=N/m  NormalDamping=P.obj.c_Table  NormalDampingUnits=N/(m/s)  NormalTransitionRegionWidth=P.bench.wContact  NormalTransitionRegionWidthUnits=m  FrictionType=SmoothStickSlip  CoefficientOfStaticFriction=P.obj.mu_s  CoefficientOfDynamicFriction=P.obj.mu_d  FrictionalCriticalVelocity=P.bench.vCrit  FrictionalCriticalVelocityUnits=m/s  SenseContactSignal=off  SensePenetrationDepth=off  SenseNormalVelocity=off  SenseTangentialVelocity=off  SensingForceTorqueDirection=BaseOnFollower  SensingForceTorqueResolutionFrame=ContactFrame  SenseNormalForce=off  SenseNormalForceMagnitude=off  SenseNormalTorque=off  SenseFrictionalForce=off  SenseFrictionalForceMagnitude=off  SenseFrictionalTorque=off  SenseTotalForce=off  SenseTotalTorque=off  SenseContactBaseRotation=off  SenseContactBaseTranslation=off  SenseContactFollowerRotation=off  SenseContactFollowerTranslation=off  ZeroCrossDetectContactStartAndEnd=off
  WallContactW : sm_lib/Forces and Torques/Spatial Contact Force  SenseSeparationDistance=off  NormalForceType=SmoothSpringDamper  NormalStiffness=P.obj.k_Table  NormalStiffnessUnits=N/m  NormalDamping=P.obj.c_Table  NormalDampingUnits=N/(m/s)  NormalTransitionRegionWidth=P.bench.wContact  NormalTransitionRegionWidthUnits=m  FrictionType=SmoothStickSlip  CoefficientOfStaticFriction=P.obj.mu_s  CoefficientOfDynamicFriction=P.obj.mu_d  FrictionalCriticalVelocity=P.bench.vCrit  FrictionalCriticalVelocityUnits=m/s  SenseContactSignal=off  SensePenetrationDepth=off  SenseNormalVelocity=off  SenseTangentialVelocity=off  SensingForceTorqueDirection=BaseOnFollower  SensingForceTorqueResolutionFrame=ContactFrame  SenseNormalForce=off  SenseNormalForceMagnitude=off  SenseNormalTorque=off  SenseFrictionalForce=off  SenseFrictionalForceMagnitude=off  SenseFrictionalTorque=off  SenseTotalForce=off  SenseTotalTorque=off  SenseContactBaseRotation=off  SenseContactBaseTranslation=off  SenseContactFollowerRotation=off  SenseContactFollowerTranslation=off  ZeroCrossDetectContactStartAndEnd=off
  WallE : sm_lib/Body Elements/Brick Solid  BrickDimensions=[P.scene.tWall P.scene.wTray P.scene.hWall]  BrickDimensionsUnits=m  ExportEntireGeometry=on  InertiaType=CalculateFromGeometry  BasedOnType=Density  Density=1000  DensityUnits=kg/m^3  Mass=1  MassUnits=kg  CenterOfMass=[0 0 0]  CenterOfMassUnits=m  MomentsOfInertia=[1 1 1]  MomentsOfInertiaUnits=kg*m^2  ProductsOfInertia=[0 0 0]  ProductsOfInertiaUnits=kg*m^2  GraphicType=FromGeometry  MarkerShape=Sphere  MarkerSize=10  GraphicVisPropType=SimpleVisualProperties  GraphicDiffuseColor=[0.2 0.35 0.6]  GraphicOpacity=1  GraphicSpecularColor=[0.5 0.5 0.5 1.0]  GraphicAmbientColor=[0.15 0.15 0.15 1.0]  GraphicEmissiveColor=[0.0 0.0 0.0 1.0]  GraphicShininess=75  DoExposeReferenceFrame=on  SerializedFrames=<Frames/>
  WallN : sm_lib/Body Elements/Brick Solid  BrickDimensions=[P.scene.wTray P.scene.tWall P.scene.hWall]  BrickDimensionsUnits=m  ExportEntireGeometry=on  InertiaType=CalculateFromGeometry  BasedOnType=Density  Density=1000  DensityUnits=kg/m^3  Mass=1  MassUnits=kg  CenterOfMass=[0 0 0]  CenterOfMassUnits=m  MomentsOfInertia=[1 1 1]  MomentsOfInertiaUnits=kg*m^2  ProductsOfInertia=[0 0 0]  ProductsOfInertiaUnits=kg*m^2  GraphicType=FromGeometry  MarkerShape=Sphere  MarkerSize=10  GraphicVisPropType=SimpleVisualProperties  GraphicDiffuseColor=[0.2 0.35 0.6]  GraphicOpacity=1  GraphicSpecularColor=[0.5 0.5 0.5 1.0]  GraphicAmbientColor=[0.15 0.15 0.15 1.0]  GraphicEmissiveColor=[0.0 0.0 0.0 1.0]  GraphicShininess=75  DoExposeReferenceFrame=on  SerializedFrames=<Frames/>
  WallPoseE : sm_lib/Frames and Transforms/Rigid Transform  RotationMethod=None  FollAlignAxisA=+X  BaseAlignAxisA=+Y  FollAlignAxisB=+Y  BaseAlignAxisB=+Z  RotationStandardAxis=+Z  RotationAngle=0  RotationAngleUnits=deg  RotationArbitraryAxis=[0 0 1]  RotationSequenceAxes=FollowerAxes  RotationSequence=XYX  RotationSequenceAngles=[0 0 0]  RotationSequenceAnglesUnits=deg  RotationMatrix=[1 0 0;0 1 0;0 0 1]  Quaternion=[1 0 0 0]  TranslationMethod=Cartesian  TranslationCartesianOffset=[P.scene.trayXY + [P.scene.wTray/2 0] P.scene.trayZ + P.scene.hWall/2]  TranslationCartesianOffsetUnits=m  TranslationStandardAxis=+Z  TranslationStandardOffset=0  TranslationStandardOffsetUnits=m  TranslationROffset=0  TranslationROffsetUnits=m  TranslationThetaOffset=0  TranslationThetaOffsetUnits=deg  TranslationZOffset=0  TranslationZOffsetUnits=m
  WallPoseN : sm_lib/Frames and Transforms/Rigid Transform  RotationMethod=None  FollAlignAxisA=+X  BaseAlignAxisA=+Y  FollAlignAxisB=+Y  BaseAlignAxisB=+Z  RotationStandardAxis=+Z  RotationAngle=0  RotationAngleUnits=deg  RotationArbitraryAxis=[0 0 1]  RotationSequenceAxes=FollowerAxes  RotationSequence=XYX  RotationSequenceAngles=[0 0 0]  RotationSequenceAnglesUnits=deg  RotationMatrix=[1 0 0;0 1 0;0 0 1]  Quaternion=[1 0 0 0]  TranslationMethod=Cartesian  TranslationCartesianOffset=[P.scene.trayXY + [0 P.scene.wTray/2] P.scene.trayZ + P.scene.hWall/2]  TranslationCartesianOffsetUnits=m  TranslationStandardAxis=+Z  TranslationStandardOffset=0  TranslationStandardOffsetUnits=m  TranslationROffset=0  TranslationROffsetUnits=m  TranslationThetaOffset=0  TranslationThetaOffsetUnits=deg  TranslationZOffset=0  TranslationZOffsetUnits=m
  WallPoseS : sm_lib/Frames and Transforms/Rigid Transform  RotationMethod=None  FollAlignAxisA=+X  BaseAlignAxisA=+Y  FollAlignAxisB=+Y  BaseAlignAxisB=+Z  RotationStandardAxis=+Z  RotationAngle=0  RotationAngleUnits=deg  RotationArbitraryAxis=[0 0 1]  RotationSequenceAxes=FollowerAxes  RotationSequence=XYX  RotationSequenceAngles=[0 0 0]  RotationSequenceAnglesUnits=deg  RotationMatrix=[1 0 0;0 1 0;0 0 1]  Quaternion=[1 0 0 0]  TranslationMethod=Cartesian  TranslationCartesianOffset=[P.scene.trayXY - [0 P.scene.wTray/2] P.scene.trayZ + P.scene.hWall/2]  TranslationCartesianOffsetUnits=m  TranslationStandardAxis=+Z  TranslationStandardOffset=0  TranslationStandardOffsetUnits=m  TranslationROffset=0  TranslationROffsetUnits=m  TranslationThetaOffset=0  TranslationThetaOffsetUnits=deg  TranslationZOffset=0  TranslationZOffsetUnits=m
  WallPoseW : sm_lib/Frames and Transforms/Rigid Transform  RotationMethod=None  FollAlignAxisA=+X  BaseAlignAxisA=+Y  FollAlignAxisB=+Y  BaseAlignAxisB=+Z  RotationStandardAxis=+Z  RotationAngle=0  RotationAngleUnits=deg  RotationArbitraryAxis=[0 0 1]  RotationSequenceAxes=FollowerAxes  RotationSequence=XYX  RotationSequenceAngles=[0 0 0]  RotationSequenceAnglesUnits=deg  RotationMatrix=[1 0 0;0 1 0;0 0 1]  Quaternion=[1 0 0 0]  TranslationMethod=Cartesian  TranslationCartesianOffset=[P.scene.trayXY - [P.scene.wTray/2 0] P.scene.trayZ + P.scene.hWall/2]  TranslationCartesianOffsetUnits=m  TranslationStandardAxis=+Z  TranslationStandardOffset=0  TranslationStandardOffsetUnits=m  TranslationROffset=0  TranslationROffsetUnits=m  TranslationThetaOffset=0  TranslationThetaOffsetUnits=deg  TranslationZOffset=0  TranslationZOffsetUnits=m
  WallS : sm_lib/Body Elements/Brick Solid  BrickDimensions=[P.scene.wTray P.scene.tWall P.scene.hWall]  BrickDimensionsUnits=m  ExportEntireGeometry=on  InertiaType=CalculateFromGeometry  BasedOnType=Density  Density=1000  DensityUnits=kg/m^3  Mass=1  MassUnits=kg  CenterOfMass=[0 0 0]  CenterOfMassUnits=m  MomentsOfInertia=[1 1 1]  MomentsOfInertiaUnits=kg*m^2  ProductsOfInertia=[0 0 0]  ProductsOfInertiaUnits=kg*m^2  GraphicType=FromGeometry  MarkerShape=Sphere  MarkerSize=10  GraphicVisPropType=SimpleVisualProperties  GraphicDiffuseColor=[0.2 0.35 0.6]  GraphicOpacity=1  GraphicSpecularColor=[0.5 0.5 0.5 1.0]  GraphicAmbientColor=[0.15 0.15 0.15 1.0]  GraphicEmissiveColor=[0.0 0.0 0.0 1.0]  GraphicShininess=75  DoExposeReferenceFrame=on  SerializedFrames=<Frames/>
  WallW : sm_lib/Body Elements/Brick Solid  BrickDimensions=[P.scene.tWall P.scene.wTray P.scene.hWall]  BrickDimensionsUnits=m  ExportEntireGeometry=on  InertiaType=CalculateFromGeometry  BasedOnType=Density  Density=1000  DensityUnits=kg/m^3  Mass=1  MassUnits=kg  CenterOfMass=[0 0 0]  CenterOfMassUnits=m  MomentsOfInertia=[1 1 1]  MomentsOfInertiaUnits=kg*m^2  ProductsOfInertia=[0 0 0]  ProductsOfInertiaUnits=kg*m^2  GraphicType=FromGeometry  MarkerShape=Sphere  MarkerSize=10  GraphicVisPropType=SimpleVisualProperties  GraphicDiffuseColor=[0.2 0.35 0.6]  GraphicOpacity=1  GraphicSpecularColor=[0.5 0.5 0.5 1.0]  GraphicAmbientColor=[0.15 0.15 0.15 1.0]  GraphicEmissiveColor=[0.0 0.0 0.0 1.0]  GraphicShininess=75  DoExposeReferenceFrame=on  SerializedFrames=<Frames/>
  World : PMIOPort  Side=Left
  ObjGeo : PMIOPort  Port=2  Side=Right
  objPose : Outport
  objState : Outport  Port=2
  wires:
  StemIntact/1 -> StemIntactSat/1
  StemIntactNeg/1 -> StemIntact/1
  StemBroken/1 -> StemIntactNeg/1
  StemBreakRate/1 -> StemBroken/1
  StemOverloadD/1 -> StemBreakRate/1
  StemOverload/1 -> StemOverloadD/1
  StemDetachSq/1 -> StemOverload/2
  StemForceSqSum/1 -> StemOverload/1
  StemForceSq/1 -> StemForceSqSum/1
  StemLagRate/1 -> StemLag/1
  StemLagErr/1 -> StemLagRate/1
  StemLag/1 -> StemLagErr/2, PS_fStem/1
  StemGate/1 -> StemLagErr/1
  StemIntactSat/1 -> StemGate/2
  StemForce/1 -> StemGate/1, StemForceSq/1
  StemC/1 -> StemForce/2
  StemK/1 -> StemForce/1
  SL_vObj/1 -> StemC/1
  StemStretch/1 -> StemK/1
  StemAnchor/1 -> StemStretch/1
  PoseMux/1 -> objPose/1  "objPose"
  SL_angObj/1 -> PoseMux/2
  SL_pObj/1 -> StemStretch/2, PoseMux/1
  Fruit/2 -> TermVz/1
  Fruit/1 -> TermZ/1
  GndObjState_P1/1 -> objState/1
  connections:
  PS_fStem/RConn1 -- StemForceApply/LConn1
  PoseSensor/RConn4 -- SL_vObj/LConn1
  PoseSensor/RConn3 -- SL_pObj/LConn1
  WallW/LConn1 -- WallContactW/LConn1
  WallPoseW/RConn1 -- WallW/RConn1
  WallE/LConn1 -- WallContactE/LConn1
  WallPoseE/RConn1 -- WallE/RConn1
  WallS/LConn1 -- WallContactS/LConn1
  WallPoseS/RConn1 -- WallS/RConn1
  WallN/LConn1 -- WallContactN/LConn1
  WallPoseN/RConn1 -- WallN/RConn1
  TrayFloor/LConn1 -- TrayFloorContact/LConn1
  TrayFloorPose/RConn1 -- TrayFloor/RConn1
  Table/LConn1 -- TableContact/LConn1
  TablePose/RConn1 -- Table/RConn1
  PoseSensor/RConn1 -- Fruit/LConn3 -- StemForceApply/RConn1
  ObjGeo/RConn1 -- WallContactN/RConn1 -- TableContact/RConn1 -- WallContactE/RConn1 -- WallContactW/RConn1 -- TrayFloorContact/RConn1 -- WallContactS/RConn1 -- Fruit/LConn2
  Fruit/LConn1 -- WallPoseS/LConn1 -- TrayFloorPose/LConn1 -- PoseSensor/LConn1 -- WallPoseE/LConn1 -- World/RConn1 -- TablePose/LConn1 -- WallPoseN/LConn1 -- WallPoseW/LConn1
  PoseSensor/RConn2 -- SL_angObj/LConn1

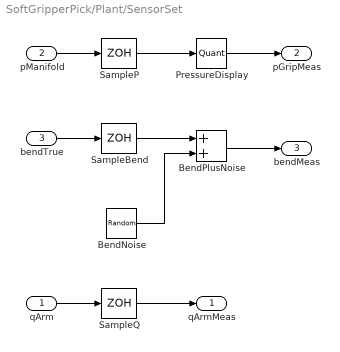
== system SoftGripperPick/Plant/SensorSet ==
  qArm : Inport
  pManifold : Inport  Port=2
  bendTrue : Inport  Port=3
  BendNoise : RandomNumber  Mean=zeros(4,1)  Variance=P.ctrl.sens.bendNoise^2  Seed=P.ctrl.sens.seed + (0:3)'  SampleTime=P.ctrl.Ts_Ctrl
  BendPlusNoise : Sum
  PressureDisplay : Quantizer  QuantizationInterval=P.ctrl.sens.pQuant
  SampleBend : ZeroOrderHold  SampleTime=P.ctrl.Ts_Ctrl
  SampleP : ZeroOrderHold  SampleTime=P.ctrl.Ts_Ctrl
  SampleQ : ZeroOrderHold  SampleTime=P.ctrl.Ts_Ctrl
  qArmMeas : Outport
  pGripMeas : Outport  Port=2
  bendMeas : Outport  Port=3
  wires:
  BendPlusNoise/1 -> bendMeas/1
  BendNoise/1 -> BendPlusNoise/2
  SampleBend/1 -> BendPlusNoise/1
  bendTrue/1 -> SampleBend/1
  PressureDisplay/1 -> pGripMeas/1
  SampleP/1 -> PressureDisplay/1
  pManifold/1 -> SampleP/1
  SampleQ/1 -> qArmMeas/1
  qArm/1 -> SampleQ/1

== system SoftGripperPick/Plant/TruthBus ==
  fContact : Inport
  objPose : Inport  Port=2
  objState : Inport  Port=3
  thetaJoints : Inport  Port=4
  pFinger : Inport  Port=5
  TruthMux : Mux  Inputs=5
  zTruth : Outport
  wires:
  TruthMux/1 -> zTruth/1
  pFinger/1 -> TruthMux/5
  thetaJoints/1 -> TruthMux/4
  objState/1 -> TruthMux/3
  objPose/1 -> TruthMux/2
  fContact/1 -> TruthMux/1
